simulink model "PMSMdetailTestbench"  (R2025b)
settings: Solver=ode1be  StartTime=0.0  StopTime=50  FixedStep=electricDrive.PmsmControlParams.Ts  RelTol=1e-3  EnableMultiTasking=on
PreLoadFcn:
  | PMSMSystemParams;
  | %PMSMthermalParams;
undefined symbols (not defined in the file or in its folder): electricDrive
libraries: fl_lib x91, nesl_utility x22, ee_lib x4, SimscapeFluids_lib x3, eeTransforms x2, simulink x2, batteryecm_lib x1, autolibshared x1, sdl_lib x1, eePmsmCurrentController x1, eePmsmFwController x1, eePmsmCurrentReferenceGen x1
(part 2 of 2)

== system PMSMdetailTestbench/Scopes/Modulation index ==
  vdq : Inport
  Vdc : Inport  Port=2
  Gain1 : Gain  Gain=1/sqrt(3)
  Math Function : Math  Operator=square  SignedPower=on
  Prevent division by 0 : Subsystem
  Product : Product  Inputs=*/
  Rate Transition4 : RateTransition  OutPortSampleTime=electricDrive.PmsmControlParams.Tsi
  Rate Transition5 : RateTransition  OutPortSampleTime=electricDrive.PmsmControlParams.Tsi
  Sqrt : Sqrt
  Sum of Elements : Sum  Inputs=+
  M : Outport  VectorParamsAs1DForOutWhenUnconnected=off
  wires:
  Sum of Elements/1 -> Sqrt/1
  Vdc/1 -> Rate Transition4/1
  Sqrt/1 -> Product/1
  Math Function/1 -> Sum of Elements/1
  Product/1 -> M/1
  Prevent division by 0/1(OUT) -> Product/2
  vdq/1 -> Rate Transition5/1
  Rate Transition4/1 -> Gain1/1
  Gain1/1 -> Prevent division by 0/1(IN)
  Rate Transition5/1 -> Math Function/1

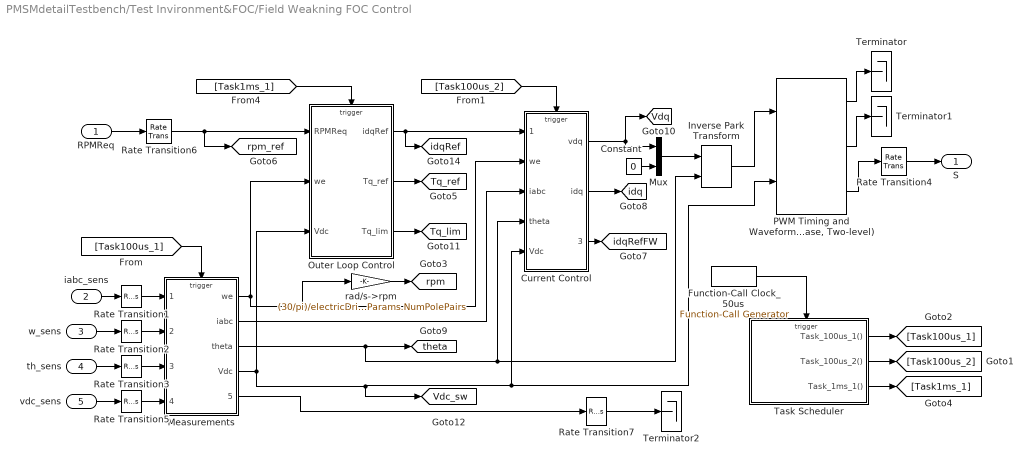
== system PMSMdetailTestbench/Test Invironment&FOC/Field Weakning FOC Control ==
  RPMReq : Inport
  iabc_sens : Inport  Port=2
  w_sens : Inport  Port=3
  th_sens : Inport  Port=4
  vdc_sens : Inport  Port=5
  Constant : Constant  Value=0  SampleTime=-1
  Current Control : Subsystem
  Function-Call Clock_50us : simulink/Ports & Subsystems/Function-Call Generator  sample_time=1e-4  numberOfIterations=1  DisallowWideOutput=off
  Inverse Park Transform : eeTransforms/Inverse Park Transform  AxisAlignment=Q-axis  PowerInvariant=off
  Measurements : Subsystem
  Mux : Mux  Inputs=2
  Outer Loop Control : Subsystem
  "PWM Timing and Waveform Generator (Three-phase, Two-level)" : eePwmGeneratorTwoLevel/PWM Timing and Waveform Generator (Three-phase, Two-level)  PWMMode=Continuous PWM (CPWM)  CPWMMode=SVM: space vector modulation  DPWMMode=60 DPWM (-30 degree shift): -30 degree shift from 60 DPWM  fsw=1e4
      settings: SamplingMode=Natural
  Rate Transition{1..7} (7 alike) : RateTransition
  Task Scheduler : Stateflow chart  TreatAsAtomicUnit=on
  Terminator : Terminator
  Terminator1 : Terminator
  Terminator2 : Terminator
  rad/s->rpm : Gain  Gain=(30/pi)/electricDrive.PmsmParams.NumPolePairs
  S : Outport  VectorParamsAs1DForOutWhenUnconnected=off
  tag scope: Tq_lim=global, Tq_ref=global, Vdc_sw=global, Vdq=global, idq=global, idqRef=global, idqRefFW=global, rpm=global, rpm_ref=global, theta=global
  wires:
  [Task100us_1] -> Measurements/Trigger
  [Task100us_2] -> Current Control/Trigger
  Current Control/1(vdq) -> Mux/1, [Vdq]
  Measurements/2(iabc) -> Current Control/3(iabc)
  Measurements/3(theta) -> Inverse Park Transform/2, Current Control/4(theta), [theta]
  Inverse Park Transform/1 -> "PWM Timing and Waveform Generator (Three-phase, Two-level)"/1
  iabc_sens/1 -> Rate Transition1/1
  w_sens/1 -> Rate Transition2/1
  th_sens/1 -> Rate Transition3/1
  vdc_sens/1 -> Rate Transition5/1
  RPMReq/1 -> Rate Transition6/1
  Rate Transition1/1 -> Measurements/1(iabc_sens)
  Rate Transition2/1 -> Measurements/2(w_sens)
  Rate Transition3/1 -> Measurements/3(th_sens)
  Rate Transition5/1 -> Measurements/4(Vdc_sens)
  Rate Transition6/1 -> [rpm_ref], Outer Loop Control/1(RPMReq)
  Measurements/4(Vdc) -> [Vdc_sw], "PWM Timing and Waveform Generator (Three-phase, Two-level)"/2, Current Control/5(Vdc), Outer Loop Control/3(Vdc)
  Function-Call Clock_50us/1 -> Task Scheduler/Trigger
  Task Scheduler/3(Task_1ms_1()) -> [Task1ms_1]
  Task Scheduler/2(Task_100us_2()) -> [Task100us_2]
  Task Scheduler/1(Task_100us_1()) -> [Task100us_1]
  Outer Loop Control/2(Tq_ref) -> [Tq_ref]
  Measurements/1(we) -> Current Control/2(we), rad/s->rpm/1, Outer Loop Control/2(we)
  rad/s->rpm/1 -> [rpm]
  Current Control/2(idq) -> [idq]
  Outer Loop Control/3(Tq_lim) -> [Tq_lim]
  Rate Transition4/1 -> S/1
  Measurements/5(PwmEnable) -> Rate Transition7/1
  [Task1ms_1] -> Outer Loop Control/Trigger
  Mux/1 -> Inverse Park Transform/1
  Constant/1 -> Mux/2
  Outer Loop Control/1(idqRef) -> Current Control/1(idq_ref), [idqRef]
  Current Control/3(idqRefFW) -> [idqRefFW]
  "PWM Timing and Waveform Generator (Three-phase, Two-level)"/1 -> Terminator/1
  "PWM Timing and Waveform Generator (Three-phase, Two-level)"/3 -> Rate Transition4/1
  "PWM Timing and Waveform Generator (Three-phase, Two-level)"/2 -> Terminator1/1
  Rate Transition7/1 -> Terminator2/1

== system PMSMdetailTestbench/Test Invironment&FOC/Motor Speed Reference ==
  VehSpd : Inport  Unit=km/hr
  Constant1 : Constant  Value=electricDrive.VehicleParams.wheel_radius
  Divide : Product  Inputs=*/
  Gain : Gain  Gain=2*pi
  Gear_ratio : Constant  Value=electricDrive.VehicleParams.Gear_ratio
  Product : Product
  Signal Specification : SignalSpecification  Unit=m/min
  Unit Conversion : UnitConversion
  MotorSpdRef : Outport  Unit=rpm  VectorParamsAs1DForOutWhenUnconnected=off
  wires:
  VehSpd/1 -> Unit Conversion/1
  Unit Conversion/1 -> Signal Specification/1
  Signal Specification/1 -> Divide/1
  Gain/1 -> Divide/2  "2*pi*R (m)"
  Divide/1 -> Product/1  "tireRpmRef"
  Gear_ratio/1 -> Product/2
  Product/1 -> MotorSpdRef/1  "motorRpmRef"
  Constant1/1 -> Gain/1  "m"

== system PMSMdetailTestbench/Test Invironment&FOC/Test Environment ==
  In1 : Inport
  Break : Constant  Value=0
  Break1 : Constant
  Bus : Subsystem
  Road Inclination : Constant
  Switch : Switch  Criteria=u2 > Threshold  Threshold=-0.4557  SaturateOnIntegerOverflow=off  InputSameDT=off
  Wind Speed : Constant  Value=0
  b : Outport
  wires:
  Wind Speed/1 -> Bus/2(Wi)
  Bus/1(b) -> b/1
  Road Inclination/1 -> Bus/1(In)
  In1/1 -> Switch/2
  Switch/1 -> Bus/3(Br)
  Break/1 -> Switch/1
  Break1/1 -> Switch/3

== system PMSMdetailTestbench/ Motor Thermal/Air_HTC_calculation/Rotor side  HTC ==
  Abs : Abs  SaturateOnIntegerOverflow=off
  Gain4 : Gain  Gain=0.75
  PS-Simulink Converter5 : nesl_utility/PS-Simulink Converter  PhysicalDomain=network_engine_domain  SubClassName=ps_output  LeftPortType=input  RightPortType=output  PseudoPeriodic=off  Frequencies=[]  VectorFormat=inherit  Unit=inherit  AffineConversion=off
  Sqrt : Sqrt
  Unit Delay3 : UnitDelay  SampleTime=-1  HasFrameUpgradeWarning=on
  RPM : PMIOPort  Side=Left
  Output : Outport
  wires:
  Gain4/1 -> Output/1
  Sqrt/1 -> Gain4/1
  Unit Delay3/1 -> Abs/1
  Abs/1 -> Sqrt/1
  PS-Simulink Converter5/1 -> Unit Delay3/1
  connections:
  RPM/RConn1 -- PS-Simulink Converter5/LConn1

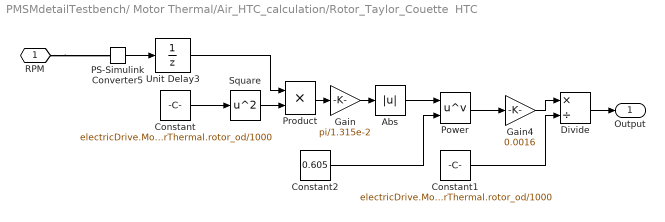
== system PMSMdetailTestbench/ Motor Thermal/Air_HTC_calculation/Rotor_Taylor_Couette  HTC ==
  Abs : Abs  SaturateOnIntegerOverflow=off
  Constant : Constant  Value=electricDrive.MotorThermal.rotor_od/1000
  Constant1 : Constant  Value=electricDrive.MotorThermal.rotor_od/1000
  Constant2 : Constant  Value=0.605
  Divide : Product  Inputs=*/
  Gain : Gain  Gain=pi/1.315e-2
  Gain4 : Gain  Gain=0.0016
  PS-Simulink Converter5 : nesl_utility/PS-Simulink Converter  PhysicalDomain=network_engine_domain  SubClassName=ps_output  LeftPortType=input  RightPortType=output  PseudoPeriodic=off  Frequencies=[]  VectorFormat=inherit  Unit=inherit  AffineConversion=off
  Power : Math  Operator=pow
  Product : Product
  Square : Math  Operator=square
  Unit Delay3 : UnitDelay  SampleTime=-1  HasFrameUpgradeWarning=on
  RPM : PMIOPort  Side=Left
  Output : Outport
  wires:
  Power/1 -> Gain4/1
  Unit Delay3/1 -> Product/1
  PS-Simulink Converter5/1 -> Unit Delay3/1
  Product/1 -> Gain/1
  Square/1 -> Product/2
  Constant/1 -> Square/1
  Gain4/1 -> Divide/1
  Constant1/1 -> Divide/2
  Divide/1 -> Output/1
  Gain/1 -> Abs/1
  Abs/1 -> Power/1
  Constant2/1 -> Power/2
  connections:
  RPM/RConn1 -- PS-Simulink Converter5/LConn1

== system PMSMdetailTestbench/ Motor Thermal/Loss Re-distribution/Iron Loss ==
  Hmot_s : Inport
  Gain1 : Gain  Gain=electricDrive.MotorThermal.vFractBridge
  Gain2 : Gain  Gain=electricDrive.MotorThermal.vFractTooth
  Unit Delay : UnitDelay  SampleTime=-1  HasFrameUpgradeWarning=on
  Unit Delay1 : UnitDelay  SampleTime=-1  HasFrameUpgradeWarning=on
  st : Outport
  rt : Outport  Port=2
  wires:
  Hmot_s/1 -> Unit Delay1/1, Unit Delay/1  "Iron_Loss"
  Gain1/1 -> rt/1
  Unit Delay/1 -> Gain2/1
  Gain2/1 -> st/1
  Unit Delay1/1 -> Gain1/1

== system PMSMdetailTestbench/ Motor Thermal/Loss Re-distribution/Subsystem ==
  Heat Flow Rate Sensor : fl_lib/Thermal/Thermal Sensors/Heat Flow Rate Sensor
  Temperature Source : fl_lib/Thermal/Thermal Sources/Temperature Source  temperature=298.15 K
  Hmot : PMIOPort  Side=Left
  Hmot_cu : PMIOPort  Port=2  Side=Right
  connections:
  Hmot_cu/RConn1 -- Heat Flow Rate Sensor/RConn1
  Hmot/RConn1 -- Heat Flow Rate Sensor/LConn1
  Temperature Source/LConn1 -- Heat Flow Rate Sensor/RConn2

== system PMSMdetailTestbench/ Motor Thermal/Loss Re-distribution/Subsystem1 ==
  Heat Flow Rate Sensor : fl_lib/Thermal/Thermal Sensors/Heat Flow Rate Sensor
  PS-Simulink Converter1 : nesl_utility/PS-Simulink Converter  PhysicalDomain=network_engine_domain  SubClassName=ps_output  LeftPortType=input  RightPortType=output  PseudoPeriodic=off  Frequencies=[]  VectorFormat=inherit  Unit=inherit  AffineConversion=off
  Temperature Source : fl_lib/Thermal/Thermal Sources/Temperature Source  temperature=298.15 K
  Hmot : PMIOPort  Side=Left
  Hmot_Fe : Outport
  wires:
  PS-Simulink Converter1/1 -> Hmot_Fe/1
  connections:
  Heat Flow Rate Sensor/RConn1 -- PS-Simulink Converter1/LConn1
  Hmot/RConn1 -- Heat Flow Rate Sensor/LConn1
  Temperature Source/LConn1 -- Heat Flow Rate Sensor/RConn2

== system PMSMdetailTestbench/ Motor Thermal/Loss Re-distribution/Subsystem2 ==
  Heat Flow Rate Sensor : fl_lib/Thermal/Thermal Sensors/Heat Flow Rate Sensor
  Temperature Source : fl_lib/Thermal/Thermal Sources/Temperature Source  temperature=298.15 K
  Hmot : PMIOPort  Side=Left
  Hmot_cu : PMIOPort  Port=2  Side=Right
  connections:
  Hmot_cu/RConn1 -- Heat Flow Rate Sensor/RConn1
  Hmot/RConn1 -- Heat Flow Rate Sensor/LConn1
  Temperature Source/LConn1 -- Heat Flow Rate Sensor/RConn2

== system PMSMdetailTestbench/ Motor Thermal/Loss Re-distribution/Subsystem3 ==
  Heat Flow Rate Sensor : fl_lib/Thermal/Thermal Sensors/Heat Flow Rate Sensor
  Temperature Source : fl_lib/Thermal/Thermal Sources/Temperature Source  temperature=298.15 K
  Hmot : PMIOPort  Side=Left
  Hmot_Cu : PMIOPort  Port=2  Side=Right
  connections:
  Hmot_Cu/RConn1 -- Heat Flow Rate Sensor/RConn1
  Hmot/RConn1 -- Heat Flow Rate Sensor/LConn1
  Temperature Source/LConn1 -- Heat Flow Rate Sensor/RConn2

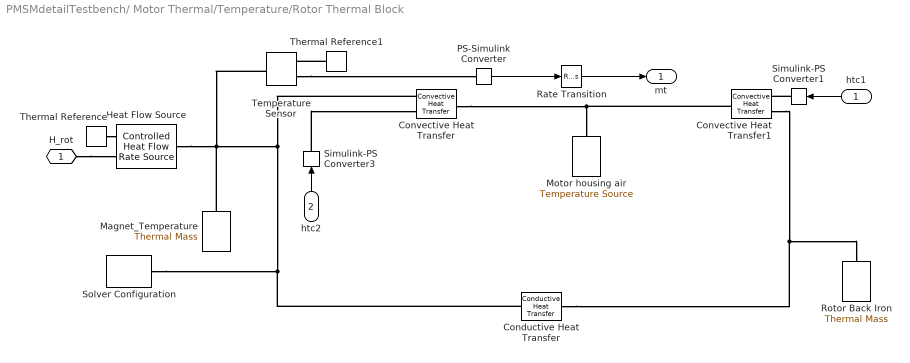
== system PMSMdetailTestbench/ Motor Thermal/Temperature/Rotor Thermal Block ==
  htc1 : Inport
  htc2 : Inport  Port=2
  Conductive Heat Transfer : fl_lib/Thermal/Thermal Elements/Conductive Heat Transfer  thermal_type=foundation.enum.ConstantVariableTabulated.Constant  wall_geometry=foundation.enum.ConductionWallGeometry.Cylindrical  area=1e-4 m^2  thickness=0.1 m  d_in=0.005 m  d_out=electricDrive.MotorThermal.rotor_od m  L=electricDrive.MotorThermal.rotorStackLength m  th_cond_min=10 W/(K*m)  th_cond=electricDrive.IronThConductivity W/(K*m)  th_cond_TLU=[413, 401, 392, 383, 371, 357, 342] W/(K*m)  temp_TLU=[200, 273, 400, 600, 800, 1000, 1200] K  T_specify=off  T_priority=None  T=0 K  T_nominal_specify=off  T_nominal_value=1  T_nominal_unit=K  Q_specify=off  Q_priority=None  Q=0 W  Q_nominal_specify=off  Q_nominal_value=1  Q_nominal_unit=W
  Convective Heat Transfer : fl_lib/Thermal/Thermal Elements/Convective Heat Transfer  thermal_type=foundation.enum.constant_variable.variable  area=electricDrive.MotorThermal.RotorAreaCyl m^2  heat_tr_coeff=10 W/(K*m^2)  min_heat_tr_coeff=1e-3 W/(K*m^2)  T_specify=off  T_priority=None  T=0 K  T_nominal_specify=off  T_nominal_value=1  T_nominal_unit=K  Q_specify=off  Q_priority=None  Q=0 W  Q_nominal_specify=off  Q_nominal_value=1  Q_nominal_unit=W
      settings: InternalSimscapePortConfiguration="{\"Bottom\":[],\"Left\":[{\"id\":\"A\",\"label\":\"A\",\"type\":\"foundation.thermal.thermal\"},{\"id\":\"var_heat_tr_coeff\",\"label\":\"K\",\"type\":\"input\"}],\"Right\":[{\"id\":\"B\",\"label\":\"B\",\"type\":\"foundation.thermal.thermal\"}],\"Top\":[]}"
  Convective Heat Transfer1 : fl_lib/Thermal/Thermal Elements/Convective Heat Transfer  thermal_type=foundation.enum.constant_variable.variable  area=electricDrive.MotorThermal.RotorAreaER m^2  heat_tr_coeff=20 W/(K*m^2)  min_heat_tr_coeff=1e-3 W/(K*m^2)  T_specify=off  T_priority=None  T=0 K  T_nominal_specify=off  T_nominal_value=1  T_nominal_unit=K  Q_specify=off  Q_priority=None  Q=0 W  Q_nominal_specify=off  Q_nominal_value=1  Q_nominal_unit=W
      settings: InternalSimscapePortConfiguration="{\"Bottom\":[],\"Left\":[{\"id\":\"A\",\"label\":\"A\",\"type\":\"foundation.thermal.thermal\"},{\"id\":\"var_heat_tr_coeff\",\"label\":\"K\",\"type\":\"input\"}],\"Right\":[{\"id\":\"B\",\"label\":\"B\",\"type\":\"foundation.thermal.thermal\"}],\"Top\":[]}"
  Heat Flow Source : fl_lib/Thermal/Thermal Sources/Controlled Heat Flow Rate Source
  "Magnet_Temperature " : fl_lib/Thermal/Thermal Elements/Thermal Mass  mass_type=foundation.enum.constant_variable.constant  mass=electricDrive.MotorThermal.Bridgemass kg  sp_heat=447 J/(K*kg)  mass_min=1e-6 kg  num_ports=foundation.enum.numPorts2.one  m_specify=off  m_priority=High  m=1 kg  m_nominal_specify=off  m_nominal_value=1  m_nominal_unit=kg  T_specify=on  T_priority=High  T=298.15 K  T_nominal_specify=off  T_nominal_value=1  T_nominal_unit=K  Q_specify=off  Q_priority=None  Q=0 W  Q_nominal_specify=off  Q_nominal_value=1  Q_nominal_unit=W
  Motor housing air : fl_lib/Thermal/Thermal Sources/Temperature Source  temperature=298.15 K
  PS-Simulink Converter : nesl_utility/PS-Simulink Converter  PhysicalDomain=network_engine_domain  SubClassName=ps_output  LeftPortType=input  RightPortType=output  PseudoPeriodic=off  Frequencies=[]  VectorFormat=inherit  Unit=inherit  AffineConversion=on
  Rate Transition : RateTransition
  Rotor Back Iron : fl_lib/Thermal/Thermal Elements/Thermal Mass  mass_type=foundation.enum.constant_variable.constant  mass=electricDrive.MotorThermal.RotorBackIronMass kg  sp_heat=447 J/(K*kg)  mass_min=1e-6 kg  num_ports=foundation.enum.numPorts2.one  m_specify=off  m_priority=High  m=1 kg  m_nominal_specify=off  m_nominal_value=1  m_nominal_unit=kg  T_specify=on  T_priority=High  T=298.15 K  T_nominal_specify=off  T_nominal_value=1  T_nominal_unit=K  Q_specify=off  Q_priority=None  Q=0 W  Q_nominal_specify=off  Q_nominal_value=1  Q_nominal_unit=W
  Simulink-PS Converter1 : nesl_utility/Simulink-PS Converter  PhysicalDomain=network_engine_domain  SubClassName=ps_input  LeftPortType=input  RightPortType=output  PseudoPeriodic=off  Frequencies=[]  NoiseDistribution=none  NoiseParameters=[]  Unit=W/(K* m^2)  AffineConversion=off  FilteringAndDerivatives=provide  SimscapeFilterOrder=1  InputFilterTimeConstant=0.001  UdotUserProvided=0
  Simulink-PS Converter3 : nesl_utility/Simulink-PS Converter  PhysicalDomain=network_engine_domain  SubClassName=ps_input  LeftPortType=input  RightPortType=output  PseudoPeriodic=off  Frequencies=[]  NoiseDistribution=none  NoiseParameters=[]  Unit=W/(K* m^2)  AffineConversion=off  FilteringAndDerivatives=provide  SimscapeFilterOrder=1  InputFilterTimeConstant=0.001  UdotUserProvided=0
  Solver Configuration : nesl_utility/Solver Configuration  PhysicalDomain=network_engine_domain  SubClassName=solver  LeftPortType=input  RightPortType=generic  Tones=[]  Harmonics=[]  SimulateNoise=off  Profile=off  UseLocalSampling=off  EnableSwitchedLinearOptims=on  FrequencyDomain=off  UseCCode=off  RelTol=0.001  AbsTol=0.001  MinStep=1e-09  ToWorkspace=off  RevertToSquareIcSolve=off  NumHomotopyIterations=100  PhasorMode=off  PhasorModeNumHarmonics=1  ConsistencySolver=NEWTON_XTOL_AFTER_FTOL  IndexReductionMethod=DerivativeReplacement  DoDC=off  ResidualTolerance=1e-09  ConsistencyTolSource=GLOBAL  ConsistencyAbsTol=0.001  ConsistencyRelTol=0.001  ConsistencyTolFactor=0.001  UseLocalSolver=on  LocalSolverChoice=NE_BACKWARD_EULER_ADVANCER  ResolveIndetEquations=on  FunctionEvalNumThread=1  LocalSolverSampleTime=electricDrive.dt  DoFixedCost=on  MaxNonlinIter=3  MaxModeIter=2  ComputeImpulses=off  ImpulseIterations=2  LinearAlgebra=auto  LinearAlgebraNumThread=0  EquationFormulation=NE_TIME_EF  DelaysMemoryBudget=1024  AutomaticFiltering=off  FilteringTimeConstant=0.001  PartitionStorageMethod=AS_NEEDED  PartitionMemoryBudget=1024  PartitionMethod=ROBUST  MultibodyUseLocalSolver=off  MultibodyLocalSolverChoice=ODE1  MultibodyLocalSolverSampleTime=0.001
  Temperature Sensor : fl_lib/Thermal/Thermal Sensors/Temperature Sensor  temperature_measure=foundation.enum.MeasurementReference.difference
  Thermal Reference : fl_lib/Thermal/Thermal Elements/Thermal Reference
  Thermal Reference1 : fl_lib/Thermal/Thermal Elements/Thermal Reference
  H_rot : PMIOPort  Side=Right
  mt : Outport
  wires:
  htc2/1 -> Simulink-PS Converter3/1
  htc1/1 -> Simulink-PS Converter1/1
  PS-Simulink Converter/1 -> Rate Transition/1
  Rate Transition/1 -> mt/1
  connections:
  Thermal Reference/LConn1 -- Heat Flow Source/RConn2
  Conductive Heat Transfer/RConn1 -- Convective Heat Transfer1/LConn1 -- Rotor Back Iron/LConn1
  Convective Heat Transfer1/RConn1 -- Convective Heat Transfer/RConn1 -- Motor housing air/LConn1
  Heat Flow Source/LConn1 -- Temperature Sensor/LConn1 -- Conductive Heat Transfer/LConn1 -- Solver Configuration/RConn1 -- Convective Heat Transfer/LConn1 -- "Magnet_Temperature "/LConn1
  Simulink-PS Converter3/RConn1 -- Convective Heat Transfer/LConn2
  H_rot/RConn1 -- Heat Flow Source/RConn1
  Simulink-PS Converter1/RConn1 -- Convective Heat Transfer1/LConn2
  Thermal Reference1/LConn1 -- Temperature Sensor/RConn1
  Temperature Sensor/RConn2 -- PS-Simulink Converter/LConn1

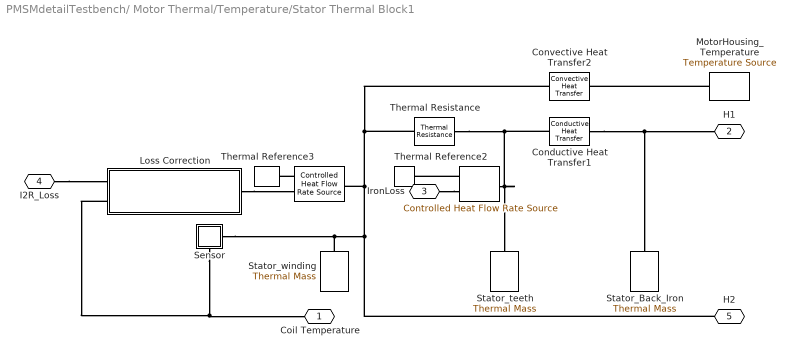
== system PMSMdetailTestbench/ Motor Thermal/Temperature/Stator Thermal Block1 ==
  " " : fl_lib/Thermal/Thermal Sources/Controlled Heat Flow Rate Source
  "  " : fl_lib/Thermal/Thermal Sources/Controlled Heat Flow Rate Source
  Conductive Heat Transfer1 : fl_lib/Thermal/Thermal Elements/Conductive Heat Transfer  thermal_type=foundation.enum.ConstantVariableTabulated.Constant  wall_geometry=foundation.enum.ConductionWallGeometry.Cylindrical  area=1e-4 m^2  thickness=0.1 m  d_in=electricDrive.MotorThermal.StatorRootDia m  d_out=electricDrive.MotorThermal.stator_od m  L=electricDrive.MotorThermal.rotorStackLength m  th_cond_min=10 W/(K*m)  th_cond=50 W/(K*m)  th_cond_TLU=[413, 401, 392, 383, 371, 357, 342] W/(K*m)  temp_TLU=[200, 273, 400, 600, 800, 1000, 1200] K  T_specify=off  T_priority=None  T=0 K  T_nominal_specify=off  T_nominal_value=1  T_nominal_unit=K  Q_specify=off  Q_priority=None  Q=0 W  Q_nominal_specify=off  Q_nominal_value=1  Q_nominal_unit=W
  Convective Heat Transfer2 : fl_lib/Thermal/Thermal Elements/Convective Heat Transfer  thermal_type=foundation.enum.constant_variable.constant  area=electricDrive.MotorThermal.StatorWindingOhArea m^2  heat_tr_coeff=1 W/(K*m^2)  min_heat_tr_coeff=1e-3 W/(K*m^2)  T_specify=off  T_priority=None  T=0 K  T_nominal_specify=off  T_nominal_value=1  T_nominal_unit=K  Q_specify=off  Q_priority=None  Q=0 W  Q_nominal_specify=off  Q_nominal_value=1  Q_nominal_unit=W
  Loss Correction : Subsystem
  MotorHousing_Temperature : fl_lib/Thermal/Thermal Sources/Temperature Source  temperature=90 degC
  Sensor : Subsystem
      settings: PortSchema="{\"entries\":[{\"content\":{\"sides\":[{\"content\":{\"connectorIds\":[\"LConn1\"]},\"type\":\"ConnectorPlacement.EquallySpacedRectSide\",\"uuid\":\"2a9c4c46-5e98-4ad3-ac1b-1643fab919e9\"},{\"content\":{\"connectorIds\":[],\"side\":\"RIGHT\"},\"type\":\"ConnectorPlacement.EquallySpacedRectSide\",\"uuid\":\"818e06c0-624d-478e-bbcc-fcb04ee6018d\"},{\"content\":{\"connectorIds\":[],\"side\":\"TOP\"},\"type\":\"ConnectorPlacement.EquallySpacedRectSide\",\"uuid\":\"5528f141-53ee-42de-bb84-2bf943b57dce\"},{\"content\":{\"connectorIds\":[\"RConn1\"],\"side\":\"BOTTOM\"},\"type\":\"ConnectorPlacement.EquallySpacedRectSide\",\"uuid\":\"84eb734e-86a3-4614-b5bf-5af47052b8ad\"}]},\"type\":\"ConnectorPlacement.EquallySpacedConnector\",\"uuid\":\"b22b55cd-2470-4ac9-8f94-59072ebe807a\"}],\"packageUris\":[\"http://schema.mathworks.com/mf0/Connector/R2020b\"],\"version\":\"1.0\"}"
  Stator_Back_Iron : fl_lib/Thermal/Thermal Elements/Thermal Mass  mass_type=foundation.enum.constant_variable.constant  mass=electricDrive.MotorThermal.StatorBackIronMass kg  sp_heat=electricDrive.IronSpHeat J/(K*kg)  mass_min=1e-6 kg  num_ports=foundation.enum.numPorts2.one  m_specify=off  m_priority=High  m=1 kg  m_nominal_specify=off  m_nominal_value=1  m_nominal_unit=kg  T_specify=off  T_priority=High  T=300 K  T_nominal_specify=off  T_nominal_value=1  T_nominal_unit=K  Q_specify=off  Q_priority=None  Q=0 W  Q_nominal_specify=off  Q_nominal_value=1  Q_nominal_unit=W
  Stator_teeth : fl_lib/Thermal/Thermal Elements/Thermal Mass  mass_type=foundation.enum.constant_variable.constant  mass=electricDrive.MotorThermal.GrossToothMass kg  sp_heat=electricDrive.IronSpHeat J/(K*kg)  mass_min=1e-6 kg  num_ports=foundation.enum.numPorts2.one  m_specify=off  m_priority=High  m=1 kg  m_nominal_specify=off  m_nominal_value=1  m_nominal_unit=kg  T_specify=off  T_priority=High  T=300 K  T_nominal_specify=off  T_nominal_value=1  T_nominal_unit=K  Q_specify=off  Q_priority=None  Q=0 W  Q_nominal_specify=off  Q_nominal_value=1  Q_nominal_unit=W
  Stator_winding : fl_lib/Thermal/Thermal Elements/Thermal Mass  mass_type=foundation.enum.constant_variable.constant  mass=electricDrive.MotorThermal.WindingMass kg  sp_heat=electricDrive.CopperSpHeat J/(K*kg)  mass_min=1e-6 kg  num_ports=foundation.enum.numPorts2.one  m_specify=off  m_priority=High  m=1 kg  m_nominal_specify=off  m_nominal_value=1  m_nominal_unit=kg  T_specify=on  T_priority=High  T=298.15 K  T_nominal_specify=off  T_nominal_value=1  T_nominal_unit=K  Q_specify=off  Q_priority=None  Q=0 W  Q_nominal_specify=off  Q_nominal_value=1  Q_nominal_unit=W
  Thermal Reference2 : fl_lib/Thermal/Thermal Elements/Thermal Reference
  Thermal Reference3 : fl_lib/Thermal/Thermal Elements/Thermal Reference
  Thermal Resistance : fl_lib/Thermal/Thermal Elements/Thermal Resistance  resistance=0.1 K/W  T_specify=off  T_priority=None  T=0 K  T_nominal_specify=off  T_nominal_value=1  T_nominal_unit=K  Q_specify=off  Q_priority=None  Q=0 W  Q_nominal_specify=off  Q_nominal_value=1  Q_nominal_unit=W
  Coil Temperature : PMIOPort  Side=Left
  H1 : PMIOPort  Port=2  Side=Left
  IronLoss : PMIOPort  Port=3  Side=Right
  I2R_Loss : PMIOPort  Port=4  Side=Right
  H2 : PMIOPort  Port=5  Side=Left
  connections:
  Conductive Heat Transfer1/RConn1 -- H1/RConn1 -- Stator_Back_Iron/LConn1
  " "/LConn1 -- Conductive Heat Transfer1/LConn1 -- Thermal Resistance/LConn1 -- Stator_teeth/LConn1
  Stator_winding/LConn1 -- H2/RConn1 -- Convective Heat Transfer2/LConn1 -- Thermal Resistance/RConn1 -- "  "/LConn1 -- Sensor/RConn1
  MotorHousing_Temperature/LConn1 -- Convective Heat Transfer2/RConn1
  "  "/RConn2 -- Thermal Reference3/LConn1
  " "/RConn2 -- Thermal Reference2/LConn1
  IronLoss/RConn1 -- " "/RConn1
  Loss Correction/RConn1 -- "  "/RConn1
  Sensor/LConn1 -- Loss Correction/LConn2 -- Coil Temperature/RConn1
  I2R_Loss/RConn1 -- Loss Correction/LConn1

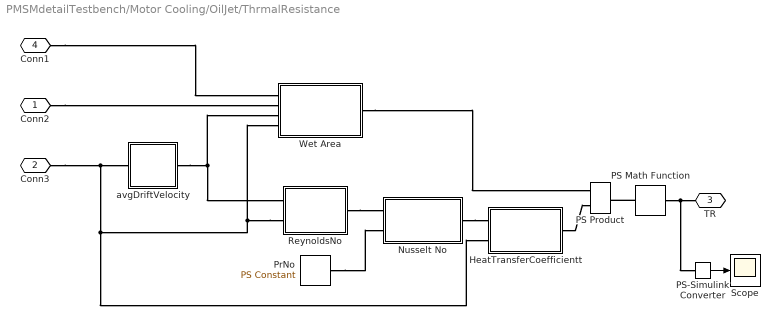
== system PMSMdetailTestbench/Motor Cooling/OilJet/ThrmalResistance  ==
  HeatTransferCoefficientt : Subsystem
  Nusselt No : Subsystem
  PS Math Function : fl_lib/Physical Signals/Functions/PS Math Function  fcn_choice=foundation.enum.math_function.reciprocal  v=1
  PS Product : fl_lib/Physical Signals/Functions/PS Product
  PS-Simulink Converter : nesl_utility/PS-Simulink Converter  PhysicalDomain=network_engine_domain  SubClassName=ps_output  LeftPortType=input  RightPortType=output  PseudoPeriodic=off  Frequencies=[]  VectorFormat=inherit  Unit=inherit  AffineConversion=off
  PrNo : fl_lib/Physical Signals/Sources/PS Constant  constant=electricDrive.MotorThermal.Pr
  ReynoldsNo : Subsystem
  Scope : Scope
  Wet Area : Subsystem
  avgDriftVelocity : Subsystem
  Conn2 : PMIOPort  Side=Left
  Conn3 : PMIOPort  Port=2  Side=Left
  TR : PMIOPort  Port=3  Side=Right
  Conn1 : PMIOPort  Port=4  Side=Right
  wires:
  PS-Simulink Converter/1 -> Scope/1
  connections:
  avgDriftVelocity/RConn1 -- ReynoldsNo/LConn1 -- Wet Area/LConn3
  ReynoldsNo/LConn2 -- Conn3/RConn1 -- avgDriftVelocity/LConn1 -- HeatTransferCoefficientt/LConn2 -- Wet Area/LConn4
  PrNo/RConn1 -- Nusselt No/LConn2
  HeatTransferCoefficientt/RConn1 -- PS Product/LConn2
  ReynoldsNo/RConn1 -- Nusselt No/LConn1
  Nusselt No/RConn1 -- HeatTransferCoefficientt/LConn1
  PS Math Function/RConn1 -- PS-Simulink Converter/LConn1 -- TR/RConn1
  Wet Area/RConn1 -- PS Product/LConn1
  PS Math Function/LConn1 -- PS Product/RConn1
  Conn1/RConn1 -- Wet Area/LConn1
  Conn2/RConn1 -- Wet Area/LConn2

== system PMSMdetailTestbench/Scopes/Modulation index/Prevent division by 0 ==
  IN : Inport
  Constant1 : Constant  Value=0.1  SampleTime=electricDrive.PmsmControlParams.Tsi
  Switch : Switch  Criteria=u2 > Threshold  Threshold=0.1  SaturateOnIntegerOverflow=off  InputSameDT=off
  OUT : Outport  VectorParamsAs1DForOutWhenUnconnected=off
  wires:
  Constant1/1 -> Switch/3
  IN/1 -> Switch/1, Switch/2
  Switch/1 -> OUT/1

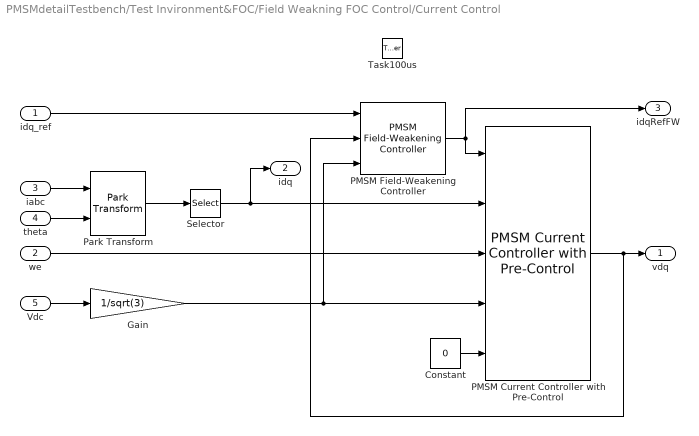
== system PMSMdetailTestbench/Test Invironment&FOC/Field Weakning FOC Control/Current Control ==
  idq_ref : Inport
  we : Inport  Port=2
  iabc : Inport  Port=3
  theta : Inport  Port=4
  Vdc : Inport  Port=5
  Task100us : TriggerPort  TriggerType=function-call  VariantControl=Variant  PortDimensions=1
  Constant : Constant  Value=0  SampleTime=-1
  Gain : Gain  Gain=1/sqrt(3)
  PMSM Current Controller with Pre-Control : eePmsmCurrentController/PMSM Current Controller with Pre-Control  Kp_id=electricDrive.PmsmControlParams.Kp_id  Ki_id=electricDrive.PmsmControlParams.Ki_id  Kaw_id=1  Kp_iq=electricDrive.PmsmControlParams.Kp_iq  Ki_iq=electricDrive.PmsmControlParams.Ki_iq  Kaw_iq=1  Ts=-1  Tsd=electricDrive.PmsmControlParams.Tsi  AxisPrio=Q-axis  ActZC=on  ActFF=on  idVect=[-200, 0, 200]  iqVect=[-200, 0, 200]  LdMatrix=electricDrive.Ld * ones(3, 3)  LqMatrix=electricDrive.Lq * ones(3, 3)  psimMatrix=electricDrive.PmsmControlParams.psim * ones(3, 3)
  PMSM Field-Weakening Controller : eePmsmFwController/PMSM Field-Weakening Controller  Mth=0.95  Kfw=electricDrive.PmsmControlParams.Ki_fw  Kaw=electricDrive.PmsmControlParams.Kaw_fw  Ts=-1
  Park Transform : eeTransforms/Park Transform  AxisAlignment=Q-axis  PowerInvariant=off
  Selector : Selector  InputPortWidth=3  IndexOptions=Index vector (dialog)  Indices=[1 2]  OutputSizes=1
  vdq : Outport  VectorParamsAs1DForOutWhenUnconnected=off
  idq : Outport  Port=2  VectorParamsAs1DForOutWhenUnconnected=off
  idqRefFW : Outport  Port=3  VectorParamsAs1DForOutWhenUnconnected=off
  wires:
  Vdc/1 -> Gain/1
  iabc/1 -> Park Transform/1
  we/1 -> PMSM Current Controller with Pre-Control/3
  theta/1 -> Park Transform/2
  Constant/1 -> PMSM Current Controller with Pre-Control/5
  Selector/1 -> PMSM Current Controller with Pre-Control/2, idq/1
  Gain/1 -> PMSM Field-Weakening Controller/3, PMSM Current Controller with Pre-Control/4
  Park Transform/1 -> Selector/1
  PMSM Field-Weakening Controller/1 -> idqRefFW/1, PMSM Current Controller with Pre-Control/1
  PMSM Current Controller with Pre-Control/1 -> PMSM Field-Weakening Controller/2, vdq/1
  idq_ref/1 -> PMSM Field-Weakening Controller/1

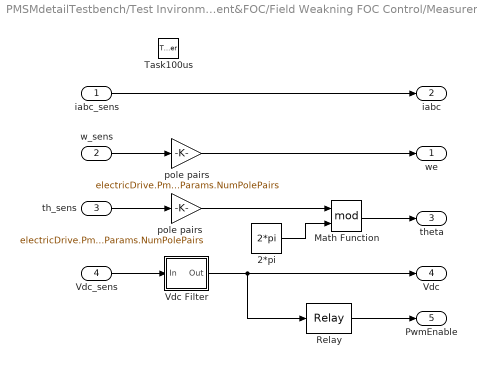
== system PMSMdetailTestbench/Test Invironment&FOC/Field Weakning FOC Control/Measurements ==
  iabc_sens : Inport
  w_sens : Inport  Port=2
  th_sens : Inport  Port=3
  Vdc_sens : Inport  Port=4
  Task100us : TriggerPort  TriggerType=function-call  VariantControl=Variant  PortDimensions=1
  2*pi : Constant  Value=2*pi  SampleTime=-1
  Math Function : Math  Operator=mod  SignedPower=on
  Relay : Relay  OnSwitchValue=200  OffSwitchValue=100
  Vdc Filter : Subsystem  mask(Discrete first-order filter (Low-pass)){T=0.005, Ts=1e-4}
      mask prompts: T "Time constant (s):"; Ts "Sample time (s):"
      mask help: This block implements a discrete low-pass filter. To calculate the coefficients, the block discretises a continuous low-pass filter using the Tustin method.
      mask init:
      | num = [ Ts/(2*T + Ts), Ts/(2*T + Ts)];
      | den = [ 1, -(2*T - Ts)/(2*T + Ts)];
  pole pairs : Gain  Gain=electricDrive.PmsmParams.NumPolePairs
  "pole pairs " : Gain  Gain=electricDrive.PmsmParams.NumPolePairs
  we : Outport  VectorParamsAs1DForOutWhenUnconnected=off
  iabc : Outport  Port=2  VectorParamsAs1DForOutWhenUnconnected=off
  theta : Outport  Port=3  VectorParamsAs1DForOutWhenUnconnected=off
  Vdc : Outport  Port=4  VectorParamsAs1DForOutWhenUnconnected=off
  PwmEnable : Outport  Port=5  VectorParamsAs1DForOutWhenUnconnected=off
  wires:
  pole pairs/1 -> we/1
  Vdc_sens/1 -> Vdc Filter/1(In)
  th_sens/1 -> "pole pairs "/1
  w_sens/1 -> pole pairs/1
  iabc_sens/1 -> iabc/1
  "pole pairs "/1 -> Math Function/1
  2*pi/1 -> Math Function/2
  Math Function/1 -> theta/1
  Relay/1 -> PwmEnable/1
  Vdc Filter/1(Out) -> Relay/1, Vdc/1

== system PMSMdetailTestbench/Test Invironment&FOC/Field Weakning FOC Control/Outer Loop Control ==
  RPMReq : Inport
  we : Inport  Port=2
  Vdc : Inport  Port=3
  Task1ms : TriggerPort  TriggerType=function-call  VariantControl=Variant  PortDimensions=1
  Constant : Constant  Value=0  SampleTime=-1
  PMSM Current Reference Generator : eePmsmCurrentReferenceGen/PMSM Current Reference Generator  Vnom=electricDrive.Vnom  Pmax=electricDrive.Pmax  Tmax=electricDrive.Tmax  Ts=-1  RefType=Zero d-axis control  rpmVec=[0, 3000]  TqVec=[-100, 0, 100]  VdcVec=[300, 350]  PWMMode=SVM: space vector modulation  ModFactor=1  idMatrix=zeros(2,3,2)  iqMatrix=zeros(2,3,2)  p=electricDrive.PmsmParams.NumPolePairs  psim=electricDrive.PmsmControlParams.psim  Ld=0.00024  Lq=0.00029  Rs=0.01  RefExpEnable=0
  Velocity Controller : eeVelocityController/Velocity Controller  CtrlType=P-PI control  Kp_w=electricDrive.PmsmControlParams.Kp_omega  Ki_w=electricDrive.PmsmControlParams.Ki_omega  Kv_w=electricDrive.PmsmControlParams.Kp_omega  Kaw_w=100  Ts=-1  Tsd=electricDrive.PmsmControlParams.Tso  ActZC=on
  elec->mech : Gain  Gain=1/electricDrive.PmsmParams.NumPolePairs
  rpm->rad/s : Gain  Gain=(pi/30)
  idqRef : Outport  VectorParamsAs1DForOutWhenUnconnected=off
  Tq_ref : Outport  Port=2  VectorParamsAs1DForOutWhenUnconnected=off
  Tq_lim : Outport  Port=3  VectorParamsAs1DForOutWhenUnconnected=off
  wires:
  rpm->rad/s/1 -> Velocity Controller/1
  Velocity Controller/1 -> PMSM Current Reference Generator/1
  RPMReq/1 -> rpm->rad/s/1
  we/1 -> elec->mech/1
  Vdc/1 -> PMSM Current Reference Generator/3
  PMSM Current Reference Generator/2 -> Tq_ref/1, Velocity Controller/3
  PMSM Current Reference Generator/3 -> Tq_lim/1
  elec->mech/1 -> PMSM Current Reference Generator/2, Velocity Controller/2
  Constant/1 -> Velocity Controller/4
  PMSM Current Reference Generator/1 -> idqRef/1

== system PMSMdetailTestbench/Test Invironment&FOC/Test Environment/Bus ==
  In : Inport
  Wi : Inport  Port=2
  Br : Inport  Port=3
  Bus Creator : BusCreator  Inputs=3
  b : Outport  VectorParamsAs1DForOutWhenUnconnected=off
  wires:
  Wi/1 -> Bus Creator/2  "Wind speed"
  Bus Creator/1 -> b/1
  Br/1 -> Bus Creator/3  "Brake pedal"
  In/1 -> Bus Creator/1  "Incline"

== system PMSMdetailTestbench/ Motor Thermal/Temperature/Stator Thermal Block1/Loss Correction ==
  PS Add : fl_lib/Physical Signals/Functions/PS Add
  PS Product : fl_lib/Physical Signals/Functions/PS Product
  PS Subtract : fl_lib/Physical Signals/Functions/PS Subtract
  Ref Temp Of loss calculations : fl_lib/Physical Signals/Sources/PS Constant  constant=298 K
  add 1 : fl_lib/Physical Signals/Sources/PS Constant  constant=1
  joule coefficient : fl_lib/Physical Signals/Functions/PS Gain  gain=0.00386 1/K
  I2R_Loss : PMIOPort  Side=Left
  Temp : PMIOPort  Port=2  Side=Left
  HCorrect : PMIOPort  Port=3  Side=Right
  connections:
  add 1/RConn1 -- PS Add/LConn2
  Ref Temp Of loss calculations/RConn1 -- PS Subtract/LConn2
  Temp/RConn1 -- PS Subtract/LConn1
  I2R_Loss/RConn1 -- PS Product/LConn2
  PS Add/RConn1 -- PS Product/LConn1
  joule coefficient/RConn1 -- PS Add/LConn1
  PS Subtract/RConn1 -- joule coefficient/LConn1
  HCorrect/RConn1 -- PS Product/RConn1

== system PMSMdetailTestbench/ Motor Thermal/Temperature/Stator Thermal Block1/Sensor ==
  Temperature Sensor : fl_lib/Thermal/Thermal Sensors/Temperature Sensor  temperature_measure=foundation.enum.MeasurementReference.difference
  Thermal Reference1 : fl_lib/Thermal/Thermal Elements/Thermal Reference
  "  " : PMIOPort  Side=Left
  " " : PMIOPort  Port=2  Side=Right
  connections:
  Thermal Reference1/LConn1 -- Temperature Sensor/RConn1
  Temperature Sensor/RConn2 -- "  "/RConn1
  " "/RConn1 -- Temperature Sensor/LConn1

== system PMSMdetailTestbench/Motor Cooling/OilJet/ThrmalResistance /HeatTransferCoefficientt ==
  PS Divide : fl_lib/Physical Signals/Functions/PS Divide
  PS Gain : fl_lib/Physical Signals/Functions/PS Gain  gain=0.126 W/(m*K)
  Conn2 : PMIOPort  Side=Left
  Conn1 : PMIOPort  Port=2  Side=Left
  Conn3 : PMIOPort  Port=3  Side=Right
  connections:
  PS Divide/LConn1 -- PS Gain/RConn1
  Conn2/RConn1 -- PS Gain/LConn1
  PS Divide/RConn1 -- Conn3/RConn1
  Conn1/RConn1 -- PS Divide/LConn2

== system PMSMdetailTestbench/Motor Cooling/OilJet/ThrmalResistance /Nusselt No ==
  PS Gain : fl_lib/Physical Signals/Functions/PS Gain  gain=0.683
  PS Math Function : fl_lib/Physical Signals/Functions/PS Math Function  fcn_choice=foundation.enum.math_function.pow  v=0.466
  PS Math Function1 : fl_lib/Physical Signals/Functions/PS Math Function  fcn_choice=foundation.enum.math_function.pow  v=1/3
  PS Product : fl_lib/Physical Signals/Functions/PS Product
  Conn1 : PMIOPort  Side=Left
  Conn2 : PMIOPort  Port=2  Side=Right
  Conn3 : PMIOPort  Port=3  Side=Left
  connections:
  PS Product/RConn1 -- Conn2/RConn1
  PS Gain/RConn1 -- PS Product/LConn1
  PS Math Function1/RConn1 -- PS Product/LConn2
  Conn3/RConn1 -- PS Math Function1/LConn1
  PS Math Function/RConn1 -- PS Gain/LConn1
  Conn1/RConn1 -- PS Math Function/LConn1

== system PMSMdetailTestbench/Motor Cooling/OilJet/ThrmalResistance /ReynoldsNo ==
  KinamaticVisc : fl_lib/Physical Signals/Sources/PS Constant  constant=electricDrive.MotorThermal.KinVisc*1e-6 m^2/s
  PS Divide : fl_lib/Physical Signals/Functions/PS Divide
  PS Gain : fl_lib/Physical Signals/Functions/PS Gain  gain=pi
  PS Product : fl_lib/Physical Signals/Functions/PS Product
  Conn1 : PMIOPort  Side=Left
  Conn2 : PMIOPort  Port=2  Side=Left
  Conn3 : PMIOPort  Port=3  Side=Right
  connections:
  KinamaticVisc/RConn1 -- PS Divide/LConn2
  Conn2/RConn1 -- PS Gain/LConn1
  PS Gain/RConn1 -- PS Product/LConn2
  PS Product/RConn1 -- PS Divide/LConn1
  PS Divide/RConn1 -- Conn3/RConn1
  Conn1/RConn1 -- PS Product/LConn1

== system PMSMdetailTestbench/Motor Cooling/OilJet/ThrmalResistance /Wet Area ==
  PS Divide : fl_lib/Physical Signals/Functions/PS Divide
  PS Gain : fl_lib/Physical Signals/Functions/PS Gain  gain=pi
  PS Product : fl_lib/Physical Signals/Functions/PS Product
  PS Product1 : fl_lib/Physical Signals/Functions/PS Product
  Conn1 : PMIOPort  Side=Left
  Conn2 : PMIOPort  Port=2  Side=Left
  Conn5 : PMIOPort  Port=3  Side=Left
  Conn4 : PMIOPort  Port=4  Side=Left
  Conn3 : PMIOPort  Port=5  Side=Right
  connections:
  Conn1/RConn1 -- PS Divide/LConn1
  Conn5/RConn1 -- PS Product/LConn2
  Conn2/RConn1 -- PS Product/LConn1
  PS Product1/RConn1 -- Conn3/RConn1
  PS Gain/RConn1 -- PS Product1/LConn2
  PS Product/RConn1 -- PS Divide/LConn2
  PS Divide/RConn1 -- PS Product1/LConn1
  Conn4/RConn1 -- PS Gain/LConn1

== system PMSMdetailTestbench/Motor Cooling/OilJet/ThrmalResistance /avgDriftVelocity ==
  "Jet Velocity " : fl_lib/Physical Signals/Sources/PS Constant  constant=0.5 m/s
  PS Add : fl_lib/Physical Signals/Functions/PS Add
  PS Add1 : fl_lib/Physical Signals/Functions/PS Add
  PS Gain : fl_lib/Physical Signals/Functions/PS Gain  gain=2*9.81 m/s^2
  PS Gain1 : fl_lib/Physical Signals/Functions/PS Gain  gain=0.5
  PS Math Function : fl_lib/Physical Signals/Functions/PS Math Function  fcn_choice=foundation.enum.math_function.square  v=1
  PS Math Function1 : fl_lib/Physical Signals/Functions/PS Math Function  fcn_choice=foundation.enum.math_function.sqrt  v=1
  vd : PMIOPort  Side=Right
  v : PMIOPort  Port=2  Side=Left
  connections:
  PS Gain/RConn1 -- PS Add/LConn2
  PS Math Function/RConn1 -- PS Add/LConn1
  PS Math Function1/RConn1 -- PS Add1/LConn2
  v/RConn1 -- PS Gain/LConn1
  "Jet Velocity "/RConn1 -- PS Math Function/LConn1 -- PS Add1/LConn1
  PS Add/RConn1 -- PS Math Function1/LConn1
  PS Gain1/LConn1 -- PS Add1/RConn1
  PS Gain1/RConn1 -- vd/RConn1

== system PMSMdetailTestbench/Test Invironment&FOC/Field Weakning FOC Control/Measurements/Vdc Filter ==
  In : Inport
  Discrete Transfer Fcn : DiscreteTransferFcn  Numerator=num  Denominator=den
  Out : Outport  VectorParamsAs1DForOutWhenUnconnected=off
  wires:
  Discrete Transfer Fcn/1 -> Out/1
  In/1 -> Discrete Transfer Fcn/1

== stateflow chart PMSMdetailTestbench/Test Invironment&FOC/Field Weakning FOC Control/Task Scheduler ==
  (default) -> (junction 23) : CLK_50us
  (junction 23) -> (junction 17)
  (junction 17) -> (junction 22) [order 2]
  (junction 17) -> (junction 22) [order 1] : [cnt%%2==0]{Task_100us_1;}
  (junction 22) -> (junction 18) [order 2]
  (junction 22) -> (junction 18) [order 1] : [cnt%%2==0]{Task_100us_2;}
  (junction 18) -> (junction 21) [order 1] : [cnt%%20==0]{Task_1ms_1;}
  (junction 18) -> (junction 21) [order 2]
  (junction 21) -> (junction 34) [order 2]
  (junction 21) -> (junction 16) [order 1] : [1]{cnt++;}
  data: cnt local int32
  events: Task_100us_1 output FUNCTION_CALL_EVENT; Task_100us_2 output FUNCTION_CALL_EVENT; Task_1ms_1 output FUNCTION_CALL_EVENT; CLK_50us input FUNCTION_CALL_EVENT
